simulink model "ASM_Traffic_new"  (R2024a)
settings: Solver=ode1  StartTime=SIM.tstart.v  StopTime=SIM.tend.v  FixedStep=SIM.StepSize.v  RelTol=1e-3
PostLoadFcn:
  | if any(exist('dsrtsu_mdlpostloadfcn', 'file') ~= 0), dsrtsu_mdlpostloadfcn('Execute', bdroot); end
  | try, asm_mdl_postloadfcn(bdroot, 'UpdateModel', 3600); catch, disp(lasterr); end,
InitFcn:
  | , if any(exist('rtifpga_mdlclblib', 'file') ~= 0), rtifpga_mdlclblib('Init', bdroot); end,
  | , if any(exist('dsmpb_private', 'file') ~= 0), dsmpb_private('dsmpb_mdlclblib', 'Init', bdroot); end,
undefined symbols (not defined in the file): _to_, a0b2, ASM_BrakeHydraulics_DemoSystems, ASM_VehicleDynamics_DemoSystems, b98103fe8ad365046cd0, BrakeCircuit, CPT, Crankshaft, DiscIntNeverNeededParam, dsmsi, FinalDriveAssembly, MDL, ModeSignals, Pos_BrakePedal_Maneuver, rad, RefSignals, s_to_rpm, SIM, SoftECU, Suspension, Tire, Transmission
libraries: ASM_Traffic_lib x135, simulink x100, ASM_Utils_lib x77, ASM_VehicleDynamics_lib x70, ASM_Environment_lib x22, dsmpblib x20, dsmsilib x15, MDLD_Utils_lib x10, ASM_BrakeHydraulics_lib x3
(part 54 of 63)

== system ASM_Traffic_new/VehicleDynamics/Plant/VehicleDynamics/VehicleMovement/ASMSignalCollector/Vehicle_Movement_Info_Car ==
  Reset[] : Inport
  CoGAndWheelVelocities : Inport  Port=2
  ASMBUS_VehicleDynamics_CoordinateTransformation : Inport  Port=3
  ASMBUS_VehicleDynamics_VehicleMotion : Inport  Port=4
  ASMBUS_VehicleDynamics_MassForcesAndTorques : Inport  Port=5
  ASMBUS_VehicleDynamics_VehicleMass : Inport  Port=6
  ASMBUS_VehicleDynamics_SensorMotion : Inport  Port=7
  ASMBUS_VehicleDynamics_Suspension : Inport  Port=8
  ASMBUS_VehicleDynamics_Steering : Inport  Port=9
  Accelerations : Subsystem
  Bus Selector : BusSelector  OutputSignals=GeneralizedVelocitiesDerivative.v_Vehicle_dt[x;y;z][m|s2],GeneralizedVelocitiesDerivative.w_Vehicle_dt[x;y;z][rad|s2],GeneralizedVelocitiesDerivative.q_Wheel_dt2[q1_Front;q2_Front;q1_Rear;q2_Rear][],GeneralizedVelocities.v_Vehicle[x;y;z][m|s],GeneralizedVelocities.w_Vehicle[x;y;z][rad|s],GeneralizedVelocities.q_Wheel_dt[q1_Front;q2_Front;q1_Rear;q2_Rear][],GeneralizedForcesAndTorques,GeneralizedVelocitiesDerivative
  Bus Selector1 : BusSelector  OutputSignals=VehiclePositionCoorSysE.Pos_Vehicle_CoorSys_E[x;y;z][m],VehiclePositionCoorSysE.Angle_V[Alpha;Beta;Gamma][deg],WheelPositionCoorSysE.Pos_FL_Wheels_CoorSys_E[x;y;z][m],WheelPositionCoorSysE.Pos_FR_Wheels_CoorSys_E[x;y;z][m],WheelPositionCoorSysE.Pos_RL_Wheels_CoorSys_E[x;y;z][m],WheelPositionCoorSysE.Pos_RR_Wheels_CoorSys_E[x;y;z][m],RotationMatrix_V_to_E[3x3],RotationMatrix_V_to_E_T[3x3],a_Gravity_CoorSys_V[x;y;z][m|s2]
  BusCreator2 : BusCreator  Inputs=8
  CoordinateTransformation : Subsystem
  Positions : Subsystem
  VehicleEquationOfMotion : Subsystem
  Velocities : Subsystem
  ASMSignalBus : Outport  VectorParamsAs1DForOutWhenUnconnected=off
  wires:
  Bus Selector1/1 -> Positions/3(Pos_Vehicle_CoorSys_E[x;y;z][m])  "<Pos_Vehicle_CoorSys_E[x;y;z][m]>"
  ASMBUS_VehicleDynamics_MassForcesAndTorques/1 -> BusCreator2/8, Accelerations/1(ASMBUS_VehicleDynamics_MassForcesAndTorques)
  Velocities/1(Velocities) -> Positions/1(Velocities), BusCreator2/2
  Bus Selector/3 -> Accelerations/8(q_Wheel_dt2[q1_Front;q2_Front;q1_Rear;q2_Rear][])  "<q_Wheel_dt2[q1_Front;q2_Front;q1_Rear;q2_Rear][]>"
  Bus Selector1/7 -> Positions/9(RotationMatrix_V_to_E[3x3])  "<RotationMatrix_V_to_E[3x3]>"
  Bus Selector1/9 -> Accelerations/5(a_Gravity_CoorSys_V[x;y;z][m|s2]), CoordinateTransformation/1(a_Gravity_CoorSys_V[x;y;z][m|s2])  "<a_Gravity_CoorSys_V[x;y;z][m|s2]>"
  Bus Selector1/2 -> Positions/4(Angle_V[Alpha;Beta;Gamma][deg])  "<Angle_V[Alpha;Beta;Gamma][deg]>"
  Bus Selector/2 -> Accelerations/7(w_Vehicle_dt[x;y;z][rad|s2])  "<w_Vehicle_dt[x;y;z][rad|s2]>"
  ASMBUS_VehicleDynamics_CoordinateTransformation/1 -> Bus Selector1/1
  Bus Selector/6 -> Velocities/4(q_Wheel_dt[q1_Front;q2_Front;q1_Rear;q2_Rear][])  "<q_Wheel_dt[q1_Front;q2_Front;q1_Rear;q2_Rear][]>"
  Bus Selector/7 -> VehicleEquationOfMotion/1(GeneralizedForcesAndTorques)  "<GeneralizedForcesAndTorques>"
  ASMBUS_VehicleDynamics_SensorMotion/1 -> BusCreator2/6
  Bus Selector1/5 -> Positions/7(Pos_RL_Wheels_CoorSys_E[x;y;z][m])  "<Pos_RL_Wheels_CoorSys_E[x;y;z][m]>"
  Positions/1(Positions) -> BusCreator2/3
  VehicleEquationOfMotion/1(VehicleEquationOfMotion) -> BusCreator2/4
  Accelerations/1(Accelerations) -> BusCreator2/1
  ASMBUS_VehicleDynamics_VehicleMass/1 -> BusCreator2/7, Accelerations/2(ASMBUS_VehicleDynamics_VehicleMass)
  ASMBUS_VehicleDynamics_VehicleMotion/1 -> Bus Selector/1
  Bus Selector1/4 -> Positions/6(Pos_FR_Wheels_CoorSys_E[x;y;z][m])  "<Pos_FR_Wheels_CoorSys_E[x;y;z][m]>"
  ASMBUS_VehicleDynamics_Steering/1 -> Accelerations/4(ASMBUS_VehicleDynamics_Steering)
  Bus Selector/5 -> Velocities/3(w_Vehicle[x;y;z][rad|s])  "<w_Vehicle[x;y;z][rad|s]>"
  Bus Selector/8 -> VehicleEquationOfMotion/2(GeneralizedVelocitiesDerivative)  "<GeneralizedVelocitiesDerivative>"
  CoordinateTransformation/1(CoordinateTransformation) -> BusCreator2/5
  Bus Selector/1 -> Accelerations/6(v_Vehicle_dt[x;y;z][m|s2])  "<v_Vehicle_dt[x;y;z][m|s2]>"
  BusCreator2/1 -> ASMSignalBus/1  "VehicleMovement"
  Bus Selector1/6 -> Positions/8(Pos_RR_Wheels_CoorSys_E[x;y;z][m])  "<Pos_RR_Wheels_CoorSys_E[x;y;z][m]>"
  Bus Selector1/3 -> Positions/5(Pos_FL_Wheels_CoorSys_E[x;y;z][m])  "<Pos_FL_Wheels_CoorSys_E[x;y;z][m]>"
  ASMBUS_VehicleDynamics_Suspension/1 -> Accelerations/3(ASMBUS_VehicleDynamics_Suspension)
  Reset[]/1 -> Positions/2(Reset[])
  CoGAndWheelVelocities/1 -> Velocities/1(CoGAndWheelVelocities)
  Bus Selector1/8 -> Positions/10(RotationMatrix_V_to_E_T[3x3])  "<RotationMatrix_V_to_E_T[3x3]>"
  Bus Selector/4 -> Velocities/2(v_Vehicle[x;y;z][m|s])  "<v_Vehicle[x;y;z][m|s]>"

== system ASM_Traffic_new/AnimationInterface/ANIMATION_INTERFACE/Sensors/Object_Sensor_2D_Points/Calc_Object_Sensor_2D_Points/Sensor_Points/ForIterator_Current ==
  dim_animation_point[] : Inport
  init_animation_point[] : Inport  Port=2
  num_sensor_rays[] : Inport  Port=3
  distance_sensor_out : Inport  Port=4
  angle_sensor_out : Inport  Port=5
  Add1 : Sum  Inputs=+-
  AnimationPoint_Idx : MultiPortSwitch  DataPortOrder=Zero-based contiguous  Inputs=2  zeroidx=on  SaturateOnIntegerOverflow=off  InputSameDT=off
  Assignment_Angle : Assignment  IndexOptions=Index vector (port)  Indices=1  OutputSizes=1
  Assignment_Distance : Assignment  IndexOptions=Index vector (port)  Indices=1  OutputSizes=1
  Calc_Output_Idx[] : Sum
  Calc_Saturated_Iteration_Idx : simulink/Discontinuities/Saturation Dynamic  OutMin=[]  OutMax=[]  OutDataTypeStr=Inherit: Same as second input  OutDataType=fixdt(1, 16)  OutScaling=2^-10  DoSatur=off
  Calc_Scaling_Step : Rounding  Operator=ceil
  Constant1 : Constant
  Constant2 : Constant
  Default_Idx : Constant
  Default_Value : Constant  Value=0
  Divide : Product  Inputs=*/
  For Iterator : ForIterator  ResetStates=reset  IterationSource=external  IterationLimit=36
  Iteration_Idx_LowBound : Constant
  Iteration_Idx_UpBound : MultiPortSwitch  DataPortOrder=Zero-based contiguous  Inputs=2  zeroidx=on  SaturateOnIntegerOverflow=off  InputSameDT=off
  Multiport Switch : MultiPortSwitch  DataPortOrder=Zero-based contiguous  Inputs=2  zeroidx=on  SaturateOnIntegerOverflow=off  InputSameDT=off
  Output_Idx : MultiPortSwitch  DataPortOrder=Zero-based contiguous  Inputs=2  zeroidx=on  SaturateOnIntegerOverflow=off  InputSameDT=off
  Point_Is_Unused : Constant  Value=0
  Product : Product
  Relational Operator : RelationalOperator  Operator=<=  OutDataTypeStr=boolean  InputSameDT=off
  Relational Operator1 : RelationalOperator  Operator=<  OutDataTypeStr=boolean  InputSameDT=off
  Relational Operator2 : RelationalOperator  Operator=<  OutDataTypeStr=boolean  InputSameDT=off
  Relational Operator3 : RelationalOperator  Operator=>  OutDataTypeStr=boolean  InputSameDT=off
  Saturate_to_sensor_output_dim : Saturate  UpperLimit=MDL.Traffic.Sensors.ObjectSensor2D_Calculation.Const_Sensor_Output_Dimension.v  LowerLimit=1
  Select_Angle : Selector  InputPortWidth=MDL.Traffic.Sensors.ObjectSensor2D_Calculation.Const_Sensor_Output_Dimension.v  IndexOptions=Starting index (port)  Indices=[1 3]  OutputSizes=1
  Select_Default_Angle : MultiPortSwitch  DataPortOrder=Zero-based contiguous  Inputs=2  zeroidx=on  SaturateOnIntegerOverflow=off  InputSameDT=off
  Select_Default_Distance : MultiPortSwitch  DataPortOrder=Zero-based contiguous  Inputs=2  zeroidx=on  SaturateOnIntegerOverflow=off  InputSameDT=off
  Select_Distance : Selector  InputPortWidth=MDL.Traffic.Sensors.ObjectSensor2D_Calculation.Const_Sensor_Output_Dimension.v  IndexOptions=Starting index (port)  Indices=[1 3]  OutputSizes=1
  distance_animation_point[m] : Outport  InitialOutput=0  VectorParamsAs1DForOutWhenUnconnected=off
  angle_animation_point[deg] : Outport  Port=2  InitialOutput=0  VectorParamsAs1DForOutWhenUnconnected=off
  flag_point_used[0|1] : Outport  Port=3  InitialOutput=0  VectorParamsAs1DForOutWhenUnconnected=off
  wires:
  Point_Is_Unused/1 -> Relational Operator3/2
  Saturate_to_sensor_output_dim/1 -> Relational Operator/1, Iteration_Idx_UpBound/3, Relational Operator1/1, Divide/1, Relational Operator2/1
  init_animation_point[]/1 -> Assignment_Distance/1, Assignment_Angle/1
  Assignment_Distance/1 -> distance_animation_point[m]/1, Relational Operator3/1
  Assignment_Angle/1 -> angle_animation_point[deg]/1
  angle_sensor_out/1 -> Select_Angle/1
  distance_sensor_out/1 -> Select_Distance/1
  Select_Distance/1 -> Select_Default_Distance/2
  Select_Angle/1 -> Select_Default_Angle/2
  Relational Operator/1 -> Multiport Switch/1
  Output_Idx/1 -> Multiport Switch/2
  Multiport Switch/1 -> Select_Angle/2, Select_Distance/2
  AnimationPoint_Idx/1 -> Multiport Switch/3, Assignment_Angle/3, Assignment_Distance/3
  For Iterator/1 -> Calc_Saturated_Iteration_Idx/2
  Iteration_Idx_LowBound/1 -> Calc_Saturated_Iteration_Idx/3
  Iteration_Idx_UpBound/1 -> Calc_Saturated_Iteration_Idx/1
  Relational Operator1/1 -> Iteration_Idx_UpBound/1
  Relational Operator2/1 -> AnimationPoint_Idx/1, Output_Idx/1, Select_Default_Distance/1, Select_Default_Angle/1
  Default_Idx/1 -> AnimationPoint_Idx/3, Output_Idx/3
  Calc_Output_Idx[]/1 -> Output_Idx/2, Relational Operator2/2
  Add1/1 -> Product/2
  Constant2/1 -> Calc_Output_Idx[]/2
  Product/1 -> Calc_Output_Idx[]/1
  Constant1/1 -> Add1/2
  Calc_Scaling_Step/1 -> Product/1
  Calc_Saturated_Iteration_Idx/1 -> Add1/1, AnimationPoint_Idx/2
  Divide/1 -> Calc_Scaling_Step/1
  dim_animation_point[]/1 -> For Iterator/1, Iteration_Idx_UpBound/2, Relational Operator1/2, Divide/2, Relational Operator/2
  num_sensor_rays[]/1 -> Saturate_to_sensor_output_dim/1
  Select_Default_Distance/1 -> Assignment_Distance/2
  Default_Value/1 -> Select_Default_Distance/3, Select_Default_Angle/3
  Select_Default_Angle/1 -> Assignment_Angle/2
  Relational Operator3/1 -> flag_point_used[0|1]/1

== system ASM_Traffic_new/DomainControl/DriverAssistance/Control/SoftECU_ACC/Soft_ECU_ACC/Map_Inputs/Maneuver ==
  note: Initial value is set
      | to AEBOff (3)
  ECU_Commands[] : Inport
  Reset[0|1] : Inport  Port=2
  ACC_BrakeMode_Default : Constant  Value=3
  Add : Sum  Inputs=+++
  Fcn1 : Fcn  Expr=u(1)==1020
  Fcn10 : Fcn  Expr=u(1)==1031
  Fcn2 : Fcn  Expr=u(1)==1030
  Fcn3 : Fcn  Expr=u(1)==1022
  Fcn4 : Fcn  Expr=u(1)==1021
  Fcn5 : Fcn  Expr=u(1)==1013
  Fcn6 : Fcn  Expr=u(1)==1011
  Fcn7 : Fcn  Expr=u(1)==1010
  Fcn8 : Fcn  Expr=u(1)==1012
  Fcn9 : Fcn  Expr=u(1)==1032
  Gain : Gain
  Gain1 : Gain  Gain=2
  Gain2 : Gain  Gain=3
  Logical Operator : Logic  Operator=OR  Inputs=4  AllPortsSameDT=off  OutDataTypeStr=boolean
  Memory : Memory  InitialCondition=3
  Switch : Switch  Threshold=0.5  SaturateOnIntegerOverflow=off  InputSameDT=off
  Switch1 : Switch  Threshold=0.5  SaturateOnIntegerOverflow=off  InputSameDT=off
  pos_edge_detection : Subsystem
  pos_edge_detection1 : Subsystem
  pos_edge_detection2 : Subsystem
  pos_edge_detection3 : Subsystem
  Sw_ACC_On[0Off|1On] : Outport  VectorParamsAs1DForOutWhenUnconnected=off
  Sw_ACC_Off[0Off|1On] : Outport  Port=2  VectorParamsAs1DForOutWhenUnconnected=off
  Sw_ACC_Cancel[0Off|1On] : Outport  Port=3  VectorParamsAs1DForOutWhenUnconnected=off
  Sw_ACC_Resume[0Off|1On] : Outport  Port=4  VectorParamsAs1DForOutWhenUnconnected=off
  Sw_ACC_Speed_Set[0Off|1On] : Outport  Port=5  VectorParamsAs1DForOutWhenUnconnected=off
  Sw_ACC_Speed_Increase[0Off|1On] : Outport  Port=6  VectorParamsAs1DForOutWhenUnconnected=off
  Sw_ACC_Speed_Decrease[0Off|1On] : Outport  Port=7  VectorParamsAs1DForOutWhenUnconnected=off
  Sw_ACC_BrakeMode[1Comfort|2AEBOnly|3AEBOff] : Outport  Port=8  VectorParamsAs1DForOutWhenUnconnected=off
  wires:
  ACC_BrakeMode_Default/1 -> Switch1/1
  Switch1/1 -> Switch/1
  Reset[0|1]/1 -> pos_edge_detection3/1(In1)
  Add/1 -> Switch1/3
  pos_edge_detection3/1(Out1) -> Logical Operator/4, Switch1/2
  Memory/1 -> Switch/3
  Switch/1 -> Memory/1, Sw_ACC_BrakeMode[1Comfort|2AEBOnly|3AEBOff]/1
  Logical Operator/1 -> Switch/2
  Gain/1 -> Add/1
  Gain1/1 -> Add/2
  Gain2/1 -> Add/3
  pos_edge_detection2/1(Out1) -> Logical Operator/3
  pos_edge_detection1/1(Out1) -> Logical Operator/2
  pos_edge_detection/1(Out1) -> Logical Operator/1
  Fcn2/1 -> Gain/1, pos_edge_detection2/1(In1)
  Fcn10/1 -> Gain1/1, pos_edge_detection1/1(In1)
  Fcn9/1 -> Gain2/1, pos_edge_detection/1(In1)
  ECU_Commands[]/1 -> Fcn3/1, Fcn2/1, Fcn10/1, Fcn9/1, Fcn4/1, Fcn1/1, Fcn5/1, Fcn8/1, Fcn6/1, Fcn7/1
  Fcn1/1 -> Sw_ACC_Speed_Set[0Off|1On]/1
  Fcn8/1 -> Sw_ACC_Cancel[0Off|1On]/1
  Fcn5/1 -> Sw_ACC_Resume[0Off|1On]/1
  Fcn4/1 -> Sw_ACC_Speed_Increase[0Off|1On]/1
  Fcn3/1 -> Sw_ACC_Speed_Decrease[0Off|1On]/1
  Fcn7/1 -> Sw_ACC_On[0Off|1On]/1
  Fcn6/1 -> Sw_ACC_Off[0Off|1On]/1

== system ASM_Traffic_new/Drivetrain/Plant/Drivetrain/Final_Drive_Assembly/ASMSignalCollector/Clutch_4WD/Clutch_4WD ==
  Bus Selector1 : BusSelector  OutputSignals=omega_Clutch_4WD_In[rad|s],Trq_Lock_Clutch_4WD[Nm],omega_Clutch_4WD_Out[rad|s]
  BusCreator1 : BusCreator  Inputs=3
  Out : Outport  VectorParamsAs1DForOutWhenUnconnected=off
  wires:
  Bus Selector1/2 -> BusCreator1/2  "<Trq_Lock_Clutch_4WD[Nm]>"
  [ASMBUS_Drivetrain_Clutch_4WD] -> Bus Selector1/1
  Bus Selector1/1 -> BusCreator1/1  "<omega_Clutch_4WD_In[rad|s]>"
  BusCreator1/1 -> Out/1  "Clutch_4WD"
  Bus Selector1/3 -> BusCreator1/3  "<omega_Clutch_4WD_Out[rad|s]>"

== system ASM_Traffic_new/Drivetrain/Plant/Drivetrain/Final_Drive_Assembly/ASMSignalCollector/Clutch_4WD/Dummy_Clutch_4WD ==
  BusCreator : BusCreator  Inputs=3
  Dummy_Trq_Lock_Clutch_4WD : Constant  Value=0
  Dummy_omega_Clutch_4WD_In : Constant  Value=0
  Dummy_omega_Clutch_4WD_Out : Constant  Value=0
  Out : Outport  VectorParamsAs1DForOutWhenUnconnected=off
  wires:
  Dummy_Trq_Lock_Clutch_4WD/1 -> BusCreator/2  "Trq_Lock_Clutch_4WD[Nm]"
  BusCreator/1 -> Out/1  "Clutch_4WD"
  Dummy_omega_Clutch_4WD_Out/1 -> BusCreator/3  "omega_Clutch_4WD_Out[rad|s]"
  Dummy_omega_Clutch_4WD_In/1 -> BusCreator/1  "omega_Clutch_4WD_In[rad|s]"

== system ASM_Traffic_new/Drivetrain/Plant/Drivetrain/Final_Drive_Assembly/ASMSignalCollector/Shaft_CF/Dummy_CF_Shaft ==
  BusCreator1 : BusCreator  Inputs=1
  Dummy_Trq_CF_Shaft[Nm] : Constant  Value=0
  Out : Outport  VectorParamsAs1DForOutWhenUnconnected=off
  wires:
  Dummy_Trq_CF_Shaft[Nm]/1 -> BusCreator1/1  "Trq_CF_Shaft[Nm]"
  BusCreator1/1 -> Out/1  "Shaft_CF"

== system ASM_Traffic_new/Drivetrain/Plant/Drivetrain/Final_Drive_Assembly/ASMSignalCollector/Shaft_CR/Dummy_CR_Shaft ==
  BusCreator1 : BusCreator  Inputs=1
  Dummy_Trq_CR_Shaft : Constant  Value=0
  Out : Outport  VectorParamsAs1DForOutWhenUnconnected=off
  wires:
  BusCreator1/1 -> Out/1  "Shaft_CR"
  Dummy_Trq_CR_Shaft/1 -> BusCreator1/1  "Trq_CR_Shaft[Nm]"

== system ASM_Traffic_new/Drivetrain/Plant/Drivetrain/Final_Drive_Assembly/ASMSignalCollector/Transfer_Gearbox/Dummy_Transfer_Gearbox ==
  BusCreator : BusCreator  Inputs=2
  Dummy_Trq_Cage : Constant  Value=0
  Dummy_omega_Shaft : Constant  Value=0
  Out : Outport  VectorParamsAs1DForOutWhenUnconnected=off
  wires:
  Dummy_omega_Shaft/1 -> BusCreator/2  "omega_Shaft[rad|s]"
  BusCreator/1 -> Out/1  "TransferGearbox"
  Dummy_Trq_Cage/1 -> BusCreator/1  "Trq_Cage[Nm]"

== system ASM_Traffic_new/Drivetrain/Plant/Drivetrain/Final_Drive_Assembly/ASMSignalCollector/Transfer_Gearbox/Transfer_Gearbox ==
  Bus Selector1 : BusSelector  OutputSignals=Trq_Cage[Nm],omega_Shaft[rad|s]
  BusCreator : BusCreator  Inputs=2
  Out : Outport  VectorParamsAs1DForOutWhenUnconnected=off
  wires:
  Bus Selector1/2 -> BusCreator/2  "<omega_Shaft[rad|s]>"
  Bus Selector1/1 -> BusCreator/1  "<Trq_Cage[Nm]>"
  BusCreator/1 -> Out/1  "TransferGearbox"
  [ASMBUS_Drivetrain_Transfer_Gearbox] -> Bus Selector1/1

== system ASM_Traffic_new/Environment/GroundTruth/UserInterface/PAR_Plant/Ego_Vehicle/Indicator_State[]/ASM_OSI_Mapping ==
  ASM_Vehicle_TurnLights[] : Inport
  Table_ASM_To_OSI : Lookup_n-D  NumberOfTableDimensions=1  BreakpointsForDimension1=[0,1,2,3]  Table=[2,3,4,5]  InterpMethod=Nearest  InternalRulePriority=Speed  RndMeth=Simplest
  Indicator_State[] : Outport  VectorParamsAs1DForOutWhenUnconnected=off
  wires:
  Table_ASM_To_OSI/1 -> Indicator_State[]/1
  ASM_Vehicle_TurnLights[]/1 -> Table_ASM_To_OSI/1

== system ASM_Traffic_new/Environment/GroundTruth/UserInterface/PAR_Plant/Fellow_Vehicles/Lightstates_Fellow1/Indicator_State[] ==
  Fellow_TurnLights[] : Inport
  ASM_OSI_Mapping : Subsystem
  Ext_Indicator_State[] : Constant  Value=0
  Multiport Switch : MultiPortSwitch  DataPortOrder=Zero-based contiguous  zeroidx=on  SaturateOnIntegerOverflow=off  InputSameDT=off
  Rounding Function : Rounding  Operator=round
  Saturation : Saturate  UpperLimit=2  LowerLimit=0
  Stim_Indicator_State[] : Constant  Value=0
  Sw_Indicator[0Stim|1Ext|2Mnv] : Constant  Value=2
  Indicator_State[] : Outport  VectorParamsAs1DForOutWhenUnconnected=off
  wires:
  ASM_OSI_Mapping/1(Indicator_State[]) -> Multiport Switch/4  "Mnv_Indicator_State[]"
  Stim_Indicator_State[]/1 -> Multiport Switch/2  "Stim_Indicator_State[]"
  Multiport Switch/1 -> Indicator_State[]/1  "Indicator_State[]"
  Saturation/1 -> Multiport Switch/1
  Rounding Function/1 -> Saturation/1
  Ext_Indicator_State[]/1 -> Multiport Switch/3  "Ext_Indicator_State[]"
  Fellow_TurnLights[]/1 -> ASM_OSI_Mapping/1(Fellow_TurnLights[])
  Sw_Indicator[0Stim|1Ext|2Mnv]/1 -> Rounding Function/1  "Sw_Indicator[0Stim|1Ext|2Mnv]"

== system ASM_Traffic_new/Environment/GroundTruth/UserInterface/PAR_Plant/Fellow_Vehicles/Lightstates_Fellow10/Indicator_State[] ==
  Fellow_TurnLights[] : Inport
  ASM_OSI_Mapping : Subsystem
  Ext_Indicator_State[] : Constant  Value=0
  Multiport Switch : MultiPortSwitch  DataPortOrder=Zero-based contiguous  zeroidx=on  SaturateOnIntegerOverflow=off  InputSameDT=off
  Rounding Function : Rounding  Operator=round
  Saturation : Saturate  UpperLimit=2  LowerLimit=0
  Stim_Indicator_State[] : Constant  Value=0
  Sw_Indicator[0Stim|1Ext|2Mnv] : Constant  Value=2
  Indicator_State[] : Outport  VectorParamsAs1DForOutWhenUnconnected=off
  wires:
  Sw_Indicator[0Stim|1Ext|2Mnv]/1 -> Rounding Function/1  "Sw_Indicator[0Stim|1Ext|2Mnv]"
  Fellow_TurnLights[]/1 -> ASM_OSI_Mapping/1(Fellow_TurnLights[])
  Ext_Indicator_State[]/1 -> Multiport Switch/3  "Ext_Indicator_State[]"
  Rounding Function/1 -> Saturation/1
  Saturation/1 -> Multiport Switch/1
  Multiport Switch/1 -> Indicator_State[]/1  "Indicator_State[]"
  Stim_Indicator_State[]/1 -> Multiport Switch/2  "Stim_Indicator_State[]"
  ASM_OSI_Mapping/1(Indicator_State[]) -> Multiport Switch/4  "Mnv_Indicator_State[]"

== system ASM_Traffic_new/Environment/GroundTruth/UserInterface/PAR_Plant/Fellow_Vehicles/Lightstates_Fellow11/Indicator_State[] ==
  Fellow_TurnLights[] : Inport
  ASM_OSI_Mapping : Subsystem
  Ext_Indicator_State[] : Constant  Value=0
  Multiport Switch : MultiPortSwitch  DataPortOrder=Zero-based contiguous  zeroidx=on  SaturateOnIntegerOverflow=off  InputSameDT=off
  Rounding Function : Rounding  Operator=round
  Saturation : Saturate  UpperLimit=2  LowerLimit=0
  Stim_Indicator_State[] : Constant  Value=0
  Sw_Indicator[0Stim|1Ext|2Mnv] : Constant  Value=2
  Indicator_State[] : Outport  VectorParamsAs1DForOutWhenUnconnected=off
  wires:
  ASM_OSI_Mapping/1(Indicator_State[]) -> Multiport Switch/4  "Mnv_Indicator_State[]"
  Stim_Indicator_State[]/1 -> Multiport Switch/2  "Stim_Indicator_State[]"
  Multiport Switch/1 -> Indicator_State[]/1  "Indicator_State[]"
  Saturation/1 -> Multiport Switch/1
  Rounding Function/1 -> Saturation/1
  Ext_Indicator_State[]/1 -> Multiport Switch/3  "Ext_Indicator_State[]"
  Fellow_TurnLights[]/1 -> ASM_OSI_Mapping/1(Fellow_TurnLights[])
  Sw_Indicator[0Stim|1Ext|2Mnv]/1 -> Rounding Function/1  "Sw_Indicator[0Stim|1Ext|2Mnv]"

== system ASM_Traffic_new/Environment/GroundTruth/UserInterface/PAR_Plant/Fellow_Vehicles/Lightstates_Fellow12/Indicator_State[] ==
  Fellow_TurnLights[] : Inport
  ASM_OSI_Mapping : Subsystem
  Ext_Indicator_State[] : Constant  Value=0
  Multiport Switch : MultiPortSwitch  DataPortOrder=Zero-based contiguous  zeroidx=on  SaturateOnIntegerOverflow=off  InputSameDT=off
  Rounding Function : Rounding  Operator=round
  Saturation : Saturate  UpperLimit=2  LowerLimit=0
  Stim_Indicator_State[] : Constant  Value=0
  Sw_Indicator[0Stim|1Ext|2Mnv] : Constant  Value=2
  Indicator_State[] : Outport  VectorParamsAs1DForOutWhenUnconnected=off
  wires:
  Sw_Indicator[0Stim|1Ext|2Mnv]/1 -> Rounding Function/1  "Sw_Indicator[0Stim|1Ext|2Mnv]"
  Fellow_TurnLights[]/1 -> ASM_OSI_Mapping/1(Fellow_TurnLights[])
  Ext_Indicator_State[]/1 -> Multiport Switch/3  "Ext_Indicator_State[]"
  Rounding Function/1 -> Saturation/1
  Saturation/1 -> Multiport Switch/1
  Multiport Switch/1 -> Indicator_State[]/1  "Indicator_State[]"
  Stim_Indicator_State[]/1 -> Multiport Switch/2  "Stim_Indicator_State[]"
  ASM_OSI_Mapping/1(Indicator_State[]) -> Multiport Switch/4  "Mnv_Indicator_State[]"

== system ASM_Traffic_new/Environment/GroundTruth/UserInterface/PAR_Plant/Fellow_Vehicles/Lightstates_Fellow13/Indicator_State[] ==
  Fellow_TurnLights[] : Inport
  ASM_OSI_Mapping : Subsystem
  Ext_Indicator_State[] : Constant  Value=0
  Multiport Switch : MultiPortSwitch  DataPortOrder=Zero-based contiguous  zeroidx=on  SaturateOnIntegerOverflow=off  InputSameDT=off
  Rounding Function : Rounding  Operator=round
  Saturation : Saturate  UpperLimit=2  LowerLimit=0
  Stim_Indicator_State[] : Constant  Value=0
  Sw_Indicator[0Stim|1Ext|2Mnv] : Constant  Value=2
  Indicator_State[] : Outport  VectorParamsAs1DForOutWhenUnconnected=off
  wires:
  ASM_OSI_Mapping/1(Indicator_State[]) -> Multiport Switch/4  "Mnv_Indicator_State[]"
  Stim_Indicator_State[]/1 -> Multiport Switch/2  "Stim_Indicator_State[]"
  Multiport Switch/1 -> Indicator_State[]/1  "Indicator_State[]"
  Saturation/1 -> Multiport Switch/1
  Rounding Function/1 -> Saturation/1
  Ext_Indicator_State[]/1 -> Multiport Switch/3  "Ext_Indicator_State[]"
  Fellow_TurnLights[]/1 -> ASM_OSI_Mapping/1(Fellow_TurnLights[])
  Sw_Indicator[0Stim|1Ext|2Mnv]/1 -> Rounding Function/1  "Sw_Indicator[0Stim|1Ext|2Mnv]"

== system ASM_Traffic_new/Environment/GroundTruth/UserInterface/PAR_Plant/Fellow_Vehicles/Lightstates_Fellow14/Indicator_State[] ==
  Fellow_TurnLights[] : Inport
  ASM_OSI_Mapping : Subsystem
  Ext_Indicator_State[] : Constant  Value=0
  Multiport Switch : MultiPortSwitch  DataPortOrder=Zero-based contiguous  zeroidx=on  SaturateOnIntegerOverflow=off  InputSameDT=off
  Rounding Function : Rounding  Operator=round
  Saturation : Saturate  UpperLimit=2  LowerLimit=0
  Stim_Indicator_State[] : Constant  Value=0
  Sw_Indicator[0Stim|1Ext|2Mnv] : Constant  Value=2
  Indicator_State[] : Outport  VectorParamsAs1DForOutWhenUnconnected=off
  wires:
  Sw_Indicator[0Stim|1Ext|2Mnv]/1 -> Rounding Function/1  "Sw_Indicator[0Stim|1Ext|2Mnv]"
  Fellow_TurnLights[]/1 -> ASM_OSI_Mapping/1(Fellow_TurnLights[])
  Ext_Indicator_State[]/1 -> Multiport Switch/3  "Ext_Indicator_State[]"
  Rounding Function/1 -> Saturation/1
  Saturation/1 -> Multiport Switch/1
  Multiport Switch/1 -> Indicator_State[]/1  "Indicator_State[]"
  Stim_Indicator_State[]/1 -> Multiport Switch/2  "Stim_Indicator_State[]"
  ASM_OSI_Mapping/1(Indicator_State[]) -> Multiport Switch/4  "Mnv_Indicator_State[]"

== system ASM_Traffic_new/Environment/GroundTruth/UserInterface/PAR_Plant/Fellow_Vehicles/Lightstates_Fellow15/Indicator_State[] ==
  Fellow_TurnLights[] : Inport
  ASM_OSI_Mapping : Subsystem
  Ext_Indicator_State[] : Constant  Value=0
  Multiport Switch : MultiPortSwitch  DataPortOrder=Zero-based contiguous  zeroidx=on  SaturateOnIntegerOverflow=off  InputSameDT=off
  Rounding Function : Rounding  Operator=round
  Saturation : Saturate  UpperLimit=2  LowerLimit=0
  Stim_Indicator_State[] : Constant  Value=0
  Sw_Indicator[0Stim|1Ext|2Mnv] : Constant  Value=2
  Indicator_State[] : Outport  VectorParamsAs1DForOutWhenUnconnected=off
  wires:
  ASM_OSI_Mapping/1(Indicator_State[]) -> Multiport Switch/4  "Mnv_Indicator_State[]"
  Stim_Indicator_State[]/1 -> Multiport Switch/2  "Stim_Indicator_State[]"
  Multiport Switch/1 -> Indicator_State[]/1  "Indicator_State[]"
  Saturation/1 -> Multiport Switch/1
  Rounding Function/1 -> Saturation/1
  Ext_Indicator_State[]/1 -> Multiport Switch/3  "Ext_Indicator_State[]"
  Fellow_TurnLights[]/1 -> ASM_OSI_Mapping/1(Fellow_TurnLights[])
  Sw_Indicator[0Stim|1Ext|2Mnv]/1 -> Rounding Function/1  "Sw_Indicator[0Stim|1Ext|2Mnv]"

== system ASM_Traffic_new/Environment/GroundTruth/UserInterface/PAR_Plant/Fellow_Vehicles/Lightstates_Fellow16/Indicator_State[] ==
  Fellow_TurnLights[] : Inport
  ASM_OSI_Mapping : Subsystem
  Ext_Indicator_State[] : Constant  Value=0
  Multiport Switch : MultiPortSwitch  DataPortOrder=Zero-based contiguous  zeroidx=on  SaturateOnIntegerOverflow=off  InputSameDT=off
  Rounding Function : Rounding  Operator=round
  Saturation : Saturate  UpperLimit=2  LowerLimit=0
  Stim_Indicator_State[] : Constant  Value=0
  Sw_Indicator[0Stim|1Ext|2Mnv] : Constant  Value=2
  Indicator_State[] : Outport  VectorParamsAs1DForOutWhenUnconnected=off
  wires:
  Sw_Indicator[0Stim|1Ext|2Mnv]/1 -> Rounding Function/1  "Sw_Indicator[0Stim|1Ext|2Mnv]"
  Fellow_TurnLights[]/1 -> ASM_OSI_Mapping/1(Fellow_TurnLights[])
  Ext_Indicator_State[]/1 -> Multiport Switch/3  "Ext_Indicator_State[]"
  Rounding Function/1 -> Saturation/1
  Saturation/1 -> Multiport Switch/1
  Multiport Switch/1 -> Indicator_State[]/1  "Indicator_State[]"
  Stim_Indicator_State[]/1 -> Multiport Switch/2  "Stim_Indicator_State[]"
  ASM_OSI_Mapping/1(Indicator_State[]) -> Multiport Switch/4  "Mnv_Indicator_State[]"

== system ASM_Traffic_new/Environment/GroundTruth/UserInterface/PAR_Plant/Fellow_Vehicles/Lightstates_Fellow17/Indicator_State[] ==
  Fellow_TurnLights[] : Inport
  ASM_OSI_Mapping : Subsystem
  Ext_Indicator_State[] : Constant  Value=0
  Multiport Switch : MultiPortSwitch  DataPortOrder=Zero-based contiguous  zeroidx=on  SaturateOnIntegerOverflow=off  InputSameDT=off
  Rounding Function : Rounding  Operator=round
  Saturation : Saturate  UpperLimit=2  LowerLimit=0
  Stim_Indicator_State[] : Constant  Value=0
  Sw_Indicator[0Stim|1Ext|2Mnv] : Constant  Value=2
  Indicator_State[] : Outport  VectorParamsAs1DForOutWhenUnconnected=off
  wires:
  ASM_OSI_Mapping/1(Indicator_State[]) -> Multiport Switch/4  "Mnv_Indicator_State[]"
  Stim_Indicator_State[]/1 -> Multiport Switch/2  "Stim_Indicator_State[]"
  Multiport Switch/1 -> Indicator_State[]/1  "Indicator_State[]"
  Saturation/1 -> Multiport Switch/1
  Rounding Function/1 -> Saturation/1
  Ext_Indicator_State[]/1 -> Multiport Switch/3  "Ext_Indicator_State[]"
  Fellow_TurnLights[]/1 -> ASM_OSI_Mapping/1(Fellow_TurnLights[])
  Sw_Indicator[0Stim|1Ext|2Mnv]/1 -> Rounding Function/1  "Sw_Indicator[0Stim|1Ext|2Mnv]"

== system ASM_Traffic_new/Environment/GroundTruth/UserInterface/PAR_Plant/Fellow_Vehicles/Lightstates_Fellow18/Indicator_State[] ==
  Fellow_TurnLights[] : Inport
  ASM_OSI_Mapping : Subsystem
  Ext_Indicator_State[] : Constant  Value=0
  Multiport Switch : MultiPortSwitch  DataPortOrder=Zero-based contiguous  zeroidx=on  SaturateOnIntegerOverflow=off  InputSameDT=off
  Rounding Function : Rounding  Operator=round
  Saturation : Saturate  UpperLimit=2  LowerLimit=0
  Stim_Indicator_State[] : Constant  Value=0
  Sw_Indicator[0Stim|1Ext|2Mnv] : Constant  Value=2
  Indicator_State[] : Outport  VectorParamsAs1DForOutWhenUnconnected=off
  wires:
  Sw_Indicator[0Stim|1Ext|2Mnv]/1 -> Rounding Function/1  "Sw_Indicator[0Stim|1Ext|2Mnv]"
  Fellow_TurnLights[]/1 -> ASM_OSI_Mapping/1(Fellow_TurnLights[])
  Ext_Indicator_State[]/1 -> Multiport Switch/3  "Ext_Indicator_State[]"
  Rounding Function/1 -> Saturation/1
  Saturation/1 -> Multiport Switch/1
  Multiport Switch/1 -> Indicator_State[]/1  "Indicator_State[]"
  Stim_Indicator_State[]/1 -> Multiport Switch/2  "Stim_Indicator_State[]"
  ASM_OSI_Mapping/1(Indicator_State[]) -> Multiport Switch/4  "Mnv_Indicator_State[]"

== system ASM_Traffic_new/Environment/GroundTruth/UserInterface/PAR_Plant/Fellow_Vehicles/Lightstates_Fellow19/Indicator_State[] ==
  Fellow_TurnLights[] : Inport
  ASM_OSI_Mapping : Subsystem
  Ext_Indicator_State[] : Constant  Value=0
  Multiport Switch : MultiPortSwitch  DataPortOrder=Zero-based contiguous  zeroidx=on  SaturateOnIntegerOverflow=off  InputSameDT=off
  Rounding Function : Rounding  Operator=round
  Saturation : Saturate  UpperLimit=2  LowerLimit=0
  Stim_Indicator_State[] : Constant  Value=0
  Sw_Indicator[0Stim|1Ext|2Mnv] : Constant  Value=2
  Indicator_State[] : Outport  VectorParamsAs1DForOutWhenUnconnected=off
  wires:
  ASM_OSI_Mapping/1(Indicator_State[]) -> Multiport Switch/4  "Mnv_Indicator_State[]"
  Stim_Indicator_State[]/1 -> Multiport Switch/2  "Stim_Indicator_State[]"
  Multiport Switch/1 -> Indicator_State[]/1  "Indicator_State[]"
  Saturation/1 -> Multiport Switch/1
  Rounding Function/1 -> Saturation/1
  Ext_Indicator_State[]/1 -> Multiport Switch/3  "Ext_Indicator_State[]"
  Fellow_TurnLights[]/1 -> ASM_OSI_Mapping/1(Fellow_TurnLights[])
  Sw_Indicator[0Stim|1Ext|2Mnv]/1 -> Rounding Function/1  "Sw_Indicator[0Stim|1Ext|2Mnv]"

== system ASM_Traffic_new/Environment/GroundTruth/UserInterface/PAR_Plant/Fellow_Vehicles/Lightstates_Fellow2/Indicator_State[] ==
  Fellow_TurnLights[] : Inport
  ASM_OSI_Mapping : Subsystem
  Ext_Indicator_State[] : Constant  Value=0
  Multiport Switch : MultiPortSwitch  DataPortOrder=Zero-based contiguous  zeroidx=on  SaturateOnIntegerOverflow=off  InputSameDT=off
  Rounding Function : Rounding  Operator=round
  Saturation : Saturate  UpperLimit=2  LowerLimit=0
  Stim_Indicator_State[] : Constant  Value=0
  Sw_Indicator[0Stim|1Ext|2Mnv] : Constant  Value=2
  Indicator_State[] : Outport  VectorParamsAs1DForOutWhenUnconnected=off
  wires:
  Sw_Indicator[0Stim|1Ext|2Mnv]/1 -> Rounding Function/1  "Sw_Indicator[0Stim|1Ext|2Mnv]"
  Fellow_TurnLights[]/1 -> ASM_OSI_Mapping/1(Fellow_TurnLights[])
  Ext_Indicator_State[]/1 -> Multiport Switch/3  "Ext_Indicator_State[]"
  Rounding Function/1 -> Saturation/1
  Saturation/1 -> Multiport Switch/1
  Multiport Switch/1 -> Indicator_State[]/1  "Indicator_State[]"
  Stim_Indicator_State[]/1 -> Multiport Switch/2  "Stim_Indicator_State[]"
  ASM_OSI_Mapping/1(Indicator_State[]) -> Multiport Switch/4  "Mnv_Indicator_State[]"

== system ASM_Traffic_new/Environment/GroundTruth/UserInterface/PAR_Plant/Fellow_Vehicles/Lightstates_Fellow20/Indicator_State[] ==
  Fellow_TurnLights[] : Inport
  ASM_OSI_Mapping : Subsystem
  Ext_Indicator_State[] : Constant  Value=0
  Multiport Switch : MultiPortSwitch  DataPortOrder=Zero-based contiguous  zeroidx=on  SaturateOnIntegerOverflow=off  InputSameDT=off
  Rounding Function : Rounding  Operator=round
  Saturation : Saturate  UpperLimit=2  LowerLimit=0
  Stim_Indicator_State[] : Constant  Value=0
  Sw_Indicator[0Stim|1Ext|2Mnv] : Constant  Value=2
  Indicator_State[] : Outport  VectorParamsAs1DForOutWhenUnconnected=off
  wires:
  Sw_Indicator[0Stim|1Ext|2Mnv]/1 -> Rounding Function/1  "Sw_Indicator[0Stim|1Ext|2Mnv]"
  Fellow_TurnLights[]/1 -> ASM_OSI_Mapping/1(Fellow_TurnLights[])
  Ext_Indicator_State[]/1 -> Multiport Switch/3  "Ext_Indicator_State[]"
  Rounding Function/1 -> Saturation/1
  Saturation/1 -> Multiport Switch/1
  Multiport Switch/1 -> Indicator_State[]/1  "Indicator_State[]"
  Stim_Indicator_State[]/1 -> Multiport Switch/2  "Stim_Indicator_State[]"
  ASM_OSI_Mapping/1(Indicator_State[]) -> Multiport Switch/4  "Mnv_Indicator_State[]"

== system ASM_Traffic_new/Environment/GroundTruth/UserInterface/PAR_Plant/Fellow_Vehicles/Lightstates_Fellow21/Indicator_State[] ==
  Fellow_TurnLights[] : Inport
  ASM_OSI_Mapping : Subsystem
  Ext_Indicator_State[] : Constant  Value=0
  Multiport Switch : MultiPortSwitch  DataPortOrder=Zero-based contiguous  zeroidx=on  SaturateOnIntegerOverflow=off  InputSameDT=off
  Rounding Function : Rounding  Operator=round
  Saturation : Saturate  UpperLimit=2  LowerLimit=0
  Stim_Indicator_State[] : Constant  Value=0
  Sw_Indicator[0Stim|1Ext|2Mnv] : Constant  Value=2
  Indicator_State[] : Outport  VectorParamsAs1DForOutWhenUnconnected=off
  wires:
  ASM_OSI_Mapping/1(Indicator_State[]) -> Multiport Switch/4  "Mnv_Indicator_State[]"
  Stim_Indicator_State[]/1 -> Multiport Switch/2  "Stim_Indicator_State[]"
  Multiport Switch/1 -> Indicator_State[]/1  "Indicator_State[]"
  Saturation/1 -> Multiport Switch/1
  Rounding Function/1 -> Saturation/1
  Ext_Indicator_State[]/1 -> Multiport Switch/3  "Ext_Indicator_State[]"
  Fellow_TurnLights[]/1 -> ASM_OSI_Mapping/1(Fellow_TurnLights[])
  Sw_Indicator[0Stim|1Ext|2Mnv]/1 -> Rounding Function/1  "Sw_Indicator[0Stim|1Ext|2Mnv]"

== system ASM_Traffic_new/Environment/GroundTruth/UserInterface/PAR_Plant/Fellow_Vehicles/Lightstates_Fellow22/Indicator_State[] ==
  Fellow_TurnLights[] : Inport
  ASM_OSI_Mapping : Subsystem
  Ext_Indicator_State[] : Constant  Value=0
  Multiport Switch : MultiPortSwitch  DataPortOrder=Zero-based contiguous  zeroidx=on  SaturateOnIntegerOverflow=off  InputSameDT=off
  Rounding Function : Rounding  Operator=round
  Saturation : Saturate  UpperLimit=2  LowerLimit=0
  Stim_Indicator_State[] : Constant  Value=0
  Sw_Indicator[0Stim|1Ext|2Mnv] : Constant  Value=2
  Indicator_State[] : Outport  VectorParamsAs1DForOutWhenUnconnected=off
  wires:
  Sw_Indicator[0Stim|1Ext|2Mnv]/1 -> Rounding Function/1  "Sw_Indicator[0Stim|1Ext|2Mnv]"
  Fellow_TurnLights[]/1 -> ASM_OSI_Mapping/1(Fellow_TurnLights[])
  Ext_Indicator_State[]/1 -> Multiport Switch/3  "Ext_Indicator_State[]"
  Rounding Function/1 -> Saturation/1
  Saturation/1 -> Multiport Switch/1
  Multiport Switch/1 -> Indicator_State[]/1  "Indicator_State[]"
  Stim_Indicator_State[]/1 -> Multiport Switch/2  "Stim_Indicator_State[]"
  ASM_OSI_Mapping/1(Indicator_State[]) -> Multiport Switch/4  "Mnv_Indicator_State[]"

== system ASM_Traffic_new/Environment/GroundTruth/UserInterface/PAR_Plant/Fellow_Vehicles/Lightstates_Fellow23/Indicator_State[] ==
  Fellow_TurnLights[] : Inport
  ASM_OSI_Mapping : Subsystem
  Ext_Indicator_State[] : Constant  Value=0
  Multiport Switch : MultiPortSwitch  DataPortOrder=Zero-based contiguous  zeroidx=on  SaturateOnIntegerOverflow=off  InputSameDT=off
  Rounding Function : Rounding  Operator=round
  Saturation : Saturate  UpperLimit=2  LowerLimit=0
  Stim_Indicator_State[] : Constant  Value=0
  Sw_Indicator[0Stim|1Ext|2Mnv] : Constant  Value=2
  Indicator_State[] : Outport  VectorParamsAs1DForOutWhenUnconnected=off
  wires:
  ASM_OSI_Mapping/1(Indicator_State[]) -> Multiport Switch/4  "Mnv_Indicator_State[]"
  Stim_Indicator_State[]/1 -> Multiport Switch/2  "Stim_Indicator_State[]"
  Multiport Switch/1 -> Indicator_State[]/1  "Indicator_State[]"
  Saturation/1 -> Multiport Switch/1
  Rounding Function/1 -> Saturation/1
  Ext_Indicator_State[]/1 -> Multiport Switch/3  "Ext_Indicator_State[]"
  Fellow_TurnLights[]/1 -> ASM_OSI_Mapping/1(Fellow_TurnLights[])
  Sw_Indicator[0Stim|1Ext|2Mnv]/1 -> Rounding Function/1  "Sw_Indicator[0Stim|1Ext|2Mnv]"

== system ASM_Traffic_new/Environment/GroundTruth/UserInterface/PAR_Plant/Fellow_Vehicles/Lightstates_Fellow24/Indicator_State[] ==
  Fellow_TurnLights[] : Inport
  ASM_OSI_Mapping : Subsystem
  Ext_Indicator_State[] : Constant  Value=0
  Multiport Switch : MultiPortSwitch  DataPortOrder=Zero-based contiguous  zeroidx=on  SaturateOnIntegerOverflow=off  InputSameDT=off
  Rounding Function : Rounding  Operator=round
  Saturation : Saturate  UpperLimit=2  LowerLimit=0
  Stim_Indicator_State[] : Constant  Value=0
  Sw_Indicator[0Stim|1Ext|2Mnv] : Constant  Value=2
  Indicator_State[] : Outport  VectorParamsAs1DForOutWhenUnconnected=off
  wires:
  Sw_Indicator[0Stim|1Ext|2Mnv]/1 -> Rounding Function/1  "Sw_Indicator[0Stim|1Ext|2Mnv]"
  Fellow_TurnLights[]/1 -> ASM_OSI_Mapping/1(Fellow_TurnLights[])
  Ext_Indicator_State[]/1 -> Multiport Switch/3  "Ext_Indicator_State[]"
  Rounding Function/1 -> Saturation/1
  Saturation/1 -> Multiport Switch/1
  Multiport Switch/1 -> Indicator_State[]/1  "Indicator_State[]"
  Stim_Indicator_State[]/1 -> Multiport Switch/2  "Stim_Indicator_State[]"
  ASM_OSI_Mapping/1(Indicator_State[]) -> Multiport Switch/4  "Mnv_Indicator_State[]"

== system ASM_Traffic_new/Environment/GroundTruth/UserInterface/PAR_Plant/Fellow_Vehicles/Lightstates_Fellow25/Indicator_State[] ==
  Fellow_TurnLights[] : Inport
  ASM_OSI_Mapping : Subsystem
  Ext_Indicator_State[] : Constant  Value=0
  Multiport Switch : MultiPortSwitch  DataPortOrder=Zero-based contiguous  zeroidx=on  SaturateOnIntegerOverflow=off  InputSameDT=off
  Rounding Function : Rounding  Operator=round
  Saturation : Saturate  UpperLimit=2  LowerLimit=0
  Stim_Indicator_State[] : Constant  Value=0
  Sw_Indicator[0Stim|1Ext|2Mnv] : Constant  Value=2
  Indicator_State[] : Outport  VectorParamsAs1DForOutWhenUnconnected=off
  wires:
  ASM_OSI_Mapping/1(Indicator_State[]) -> Multiport Switch/4  "Mnv_Indicator_State[]"
  Stim_Indicator_State[]/1 -> Multiport Switch/2  "Stim_Indicator_State[]"
  Multiport Switch/1 -> Indicator_State[]/1  "Indicator_State[]"
  Saturation/1 -> Multiport Switch/1
  Rounding Function/1 -> Saturation/1
  Ext_Indicator_State[]/1 -> Multiport Switch/3  "Ext_Indicator_State[]"
  Fellow_TurnLights[]/1 -> ASM_OSI_Mapping/1(Fellow_TurnLights[])
  Sw_Indicator[0Stim|1Ext|2Mnv]/1 -> Rounding Function/1  "Sw_Indicator[0Stim|1Ext|2Mnv]"

== system ASM_Traffic_new/Environment/GroundTruth/UserInterface/PAR_Plant/Fellow_Vehicles/Lightstates_Fellow26/Indicator_State[] ==
  Fellow_TurnLights[] : Inport
  ASM_OSI_Mapping : Subsystem
  Ext_Indicator_State[] : Constant  Value=0
  Multiport Switch : MultiPortSwitch  DataPortOrder=Zero-based contiguous  zeroidx=on  SaturateOnIntegerOverflow=off  InputSameDT=off
  Rounding Function : Rounding  Operator=round
  Saturation : Saturate  UpperLimit=2  LowerLimit=0
  Stim_Indicator_State[] : Constant  Value=0
  Sw_Indicator[0Stim|1Ext|2Mnv] : Constant  Value=2
  Indicator_State[] : Outport  VectorParamsAs1DForOutWhenUnconnected=off
  wires:
  Sw_Indicator[0Stim|1Ext|2Mnv]/1 -> Rounding Function/1  "Sw_Indicator[0Stim|1Ext|2Mnv]"
  Fellow_TurnLights[]/1 -> ASM_OSI_Mapping/1(Fellow_TurnLights[])
  Ext_Indicator_State[]/1 -> Multiport Switch/3  "Ext_Indicator_State[]"
  Rounding Function/1 -> Saturation/1
  Saturation/1 -> Multiport Switch/1
  Multiport Switch/1 -> Indicator_State[]/1  "Indicator_State[]"
  Stim_Indicator_State[]/1 -> Multiport Switch/2  "Stim_Indicator_State[]"
  ASM_OSI_Mapping/1(Indicator_State[]) -> Multiport Switch/4  "Mnv_Indicator_State[]"

== system ASM_Traffic_new/Environment/GroundTruth/UserInterface/PAR_Plant/Fellow_Vehicles/Lightstates_Fellow27/Indicator_State[] ==
  Fellow_TurnLights[] : Inport
  ASM_OSI_Mapping : Subsystem
  Ext_Indicator_State[] : Constant  Value=0
  Multiport Switch : MultiPortSwitch  DataPortOrder=Zero-based contiguous  zeroidx=on  SaturateOnIntegerOverflow=off  InputSameDT=off
  Rounding Function : Rounding  Operator=round
  Saturation : Saturate  UpperLimit=2  LowerLimit=0
  Stim_Indicator_State[] : Constant  Value=0
  Sw_Indicator[0Stim|1Ext|2Mnv] : Constant  Value=2
  Indicator_State[] : Outport  VectorParamsAs1DForOutWhenUnconnected=off
  wires:
  ASM_OSI_Mapping/1(Indicator_State[]) -> Multiport Switch/4  "Mnv_Indicator_State[]"
  Stim_Indicator_State[]/1 -> Multiport Switch/2  "Stim_Indicator_State[]"
  Multiport Switch/1 -> Indicator_State[]/1  "Indicator_State[]"
  Saturation/1 -> Multiport Switch/1
  Rounding Function/1 -> Saturation/1
  Ext_Indicator_State[]/1 -> Multiport Switch/3  "Ext_Indicator_State[]"
  Fellow_TurnLights[]/1 -> ASM_OSI_Mapping/1(Fellow_TurnLights[])
  Sw_Indicator[0Stim|1Ext|2Mnv]/1 -> Rounding Function/1  "Sw_Indicator[0Stim|1Ext|2Mnv]"

== system ASM_Traffic_new/Environment/GroundTruth/UserInterface/PAR_Plant/Fellow_Vehicles/Lightstates_Fellow28/Indicator_State[] ==
  Fellow_TurnLights[] : Inport
  ASM_OSI_Mapping : Subsystem
  Ext_Indicator_State[] : Constant  Value=0
  Multiport Switch : MultiPortSwitch  DataPortOrder=Zero-based contiguous  zeroidx=on  SaturateOnIntegerOverflow=off  InputSameDT=off
  Rounding Function : Rounding  Operator=round
  Saturation : Saturate  UpperLimit=2  LowerLimit=0
  Stim_Indicator_State[] : Constant  Value=0
  Sw_Indicator[0Stim|1Ext|2Mnv] : Constant  Value=2
  Indicator_State[] : Outport  VectorParamsAs1DForOutWhenUnconnected=off
  wires:
  Sw_Indicator[0Stim|1Ext|2Mnv]/1 -> Rounding Function/1  "Sw_Indicator[0Stim|1Ext|2Mnv]"
  Fellow_TurnLights[]/1 -> ASM_OSI_Mapping/1(Fellow_TurnLights[])
  Ext_Indicator_State[]/1 -> Multiport Switch/3  "Ext_Indicator_State[]"
  Rounding Function/1 -> Saturation/1
  Saturation/1 -> Multiport Switch/1
  Multiport Switch/1 -> Indicator_State[]/1  "Indicator_State[]"
  Stim_Indicator_State[]/1 -> Multiport Switch/2  "Stim_Indicator_State[]"
  ASM_OSI_Mapping/1(Indicator_State[]) -> Multiport Switch/4  "Mnv_Indicator_State[]"

== system ASM_Traffic_new/Environment/GroundTruth/UserInterface/PAR_Plant/Fellow_Vehicles/Lightstates_Fellow29/Indicator_State[] ==
  Fellow_TurnLights[] : Inport
  ASM_OSI_Mapping : Subsystem
  Ext_Indicator_State[] : Constant  Value=0
  Multiport Switch : MultiPortSwitch  DataPortOrder=Zero-based contiguous  zeroidx=on  SaturateOnIntegerOverflow=off  InputSameDT=off
  Rounding Function : Rounding  Operator=round
  Saturation : Saturate  UpperLimit=2  LowerLimit=0
  Stim_Indicator_State[] : Constant  Value=0
  Sw_Indicator[0Stim|1Ext|2Mnv] : Constant  Value=2
  Indicator_State[] : Outport  VectorParamsAs1DForOutWhenUnconnected=off
  wires:
  ASM_OSI_Mapping/1(Indicator_State[]) -> Multiport Switch/4  "Mnv_Indicator_State[]"
  Stim_Indicator_State[]/1 -> Multiport Switch/2  "Stim_Indicator_State[]"
  Multiport Switch/1 -> Indicator_State[]/1  "Indicator_State[]"
  Saturation/1 -> Multiport Switch/1
  Rounding Function/1 -> Saturation/1
  Ext_Indicator_State[]/1 -> Multiport Switch/3  "Ext_Indicator_State[]"
  Fellow_TurnLights[]/1 -> ASM_OSI_Mapping/1(Fellow_TurnLights[])
  Sw_Indicator[0Stim|1Ext|2Mnv]/1 -> Rounding Function/1  "Sw_Indicator[0Stim|1Ext|2Mnv]"

== system ASM_Traffic_new/Environment/GroundTruth/UserInterface/PAR_Plant/Fellow_Vehicles/Lightstates_Fellow3/Indicator_State[] ==
  Fellow_TurnLights[] : Inport
  ASM_OSI_Mapping : Subsystem
  Ext_Indicator_State[] : Constant  Value=0
  Multiport Switch : MultiPortSwitch  DataPortOrder=Zero-based contiguous  zeroidx=on  SaturateOnIntegerOverflow=off  InputSameDT=off
  Rounding Function : Rounding  Operator=round
  Saturation : Saturate  UpperLimit=2  LowerLimit=0
  Stim_Indicator_State[] : Constant  Value=0
  Sw_Indicator[0Stim|1Ext|2Mnv] : Constant  Value=2
  Indicator_State[] : Outport  VectorParamsAs1DForOutWhenUnconnected=off
  wires:
  ASM_OSI_Mapping/1(Indicator_State[]) -> Multiport Switch/4  "Mnv_Indicator_State[]"
  Stim_Indicator_State[]/1 -> Multiport Switch/2  "Stim_Indicator_State[]"
  Multiport Switch/1 -> Indicator_State[]/1  "Indicator_State[]"
  Saturation/1 -> Multiport Switch/1
  Rounding Function/1 -> Saturation/1
  Ext_Indicator_State[]/1 -> Multiport Switch/3  "Ext_Indicator_State[]"
  Fellow_TurnLights[]/1 -> ASM_OSI_Mapping/1(Fellow_TurnLights[])
  Sw_Indicator[0Stim|1Ext|2Mnv]/1 -> Rounding Function/1  "Sw_Indicator[0Stim|1Ext|2Mnv]"

== system ASM_Traffic_new/Environment/GroundTruth/UserInterface/PAR_Plant/Fellow_Vehicles/Lightstates_Fellow30/Indicator_State[] ==
  Fellow_TurnLights[] : Inport
  ASM_OSI_Mapping : Subsystem
  Ext_Indicator_State[] : Constant  Value=0
  Multiport Switch : MultiPortSwitch  DataPortOrder=Zero-based contiguous  zeroidx=on  SaturateOnIntegerOverflow=off  InputSameDT=off
  Rounding Function : Rounding  Operator=round
  Saturation : Saturate  UpperLimit=2  LowerLimit=0
  Stim_Indicator_State[] : Constant  Value=0
  Sw_Indicator[0Stim|1Ext|2Mnv] : Constant  Value=2
  Indicator_State[] : Outport  VectorParamsAs1DForOutWhenUnconnected=off
  wires:
  Sw_Indicator[0Stim|1Ext|2Mnv]/1 -> Rounding Function/1  "Sw_Indicator[0Stim|1Ext|2Mnv]"
  Fellow_TurnLights[]/1 -> ASM_OSI_Mapping/1(Fellow_TurnLights[])
  Ext_Indicator_State[]/1 -> Multiport Switch/3  "Ext_Indicator_State[]"
  Rounding Function/1 -> Saturation/1
  Saturation/1 -> Multiport Switch/1
  Multiport Switch/1 -> Indicator_State[]/1  "Indicator_State[]"
  Stim_Indicator_State[]/1 -> Multiport Switch/2  "Stim_Indicator_State[]"
  ASM_OSI_Mapping/1(Indicator_State[]) -> Multiport Switch/4  "Mnv_Indicator_State[]"

== system ASM_Traffic_new/Environment/GroundTruth/UserInterface/PAR_Plant/Fellow_Vehicles/Lightstates_Fellow4/Indicator_State[] ==
  Fellow_TurnLights[] : Inport
  ASM_OSI_Mapping : Subsystem
  Ext_Indicator_State[] : Constant  Value=0
  Multiport Switch : MultiPortSwitch  DataPortOrder=Zero-based contiguous  zeroidx=on  SaturateOnIntegerOverflow=off  InputSameDT=off
  Rounding Function : Rounding  Operator=round
  Saturation : Saturate  UpperLimit=2  LowerLimit=0
  Stim_Indicator_State[] : Constant  Value=0
  Sw_Indicator[0Stim|1Ext|2Mnv] : Constant  Value=2
  Indicator_State[] : Outport  VectorParamsAs1DForOutWhenUnconnected=off
  wires:
  Sw_Indicator[0Stim|1Ext|2Mnv]/1 -> Rounding Function/1  "Sw_Indicator[0Stim|1Ext|2Mnv]"
  Fellow_TurnLights[]/1 -> ASM_OSI_Mapping/1(Fellow_TurnLights[])
  Ext_Indicator_State[]/1 -> Multiport Switch/3  "Ext_Indicator_State[]"
  Rounding Function/1 -> Saturation/1
  Saturation/1 -> Multiport Switch/1
  Multiport Switch/1 -> Indicator_State[]/1  "Indicator_State[]"
  Stim_Indicator_State[]/1 -> Multiport Switch/2  "Stim_Indicator_State[]"
  ASM_OSI_Mapping/1(Indicator_State[]) -> Multiport Switch/4  "Mnv_Indicator_State[]"

== system ASM_Traffic_new/Environment/GroundTruth/UserInterface/PAR_Plant/Fellow_Vehicles/Lightstates_Fellow5/Indicator_State[] ==
  Fellow_TurnLights[] : Inport
  ASM_OSI_Mapping : Subsystem
  Ext_Indicator_State[] : Constant  Value=0
  Multiport Switch : MultiPortSwitch  DataPortOrder=Zero-based contiguous  zeroidx=on  SaturateOnIntegerOverflow=off  InputSameDT=off
  Rounding Function : Rounding  Operator=round
  Saturation : Saturate  UpperLimit=2  LowerLimit=0
  Stim_Indicator_State[] : Constant  Value=0
  Sw_Indicator[0Stim|1Ext|2Mnv] : Constant  Value=2
  Indicator_State[] : Outport  VectorParamsAs1DForOutWhenUnconnected=off
  wires:
  ASM_OSI_Mapping/1(Indicator_State[]) -> Multiport Switch/4  "Mnv_Indicator_State[]"
  Stim_Indicator_State[]/1 -> Multiport Switch/2  "Stim_Indicator_State[]"
  Multiport Switch/1 -> Indicator_State[]/1  "Indicator_State[]"
  Saturation/1 -> Multiport Switch/1
  Rounding Function/1 -> Saturation/1
  Ext_Indicator_State[]/1 -> Multiport Switch/3  "Ext_Indicator_State[]"
  Fellow_TurnLights[]/1 -> ASM_OSI_Mapping/1(Fellow_TurnLights[])
  Sw_Indicator[0Stim|1Ext|2Mnv]/1 -> Rounding Function/1  "Sw_Indicator[0Stim|1Ext|2Mnv]"

== system ASM_Traffic_new/Environment/GroundTruth/UserInterface/PAR_Plant/Fellow_Vehicles/Lightstates_Fellow6/Indicator_State[] ==
  Fellow_TurnLights[] : Inport
  ASM_OSI_Mapping : Subsystem
  Ext_Indicator_State[] : Constant  Value=0
  Multiport Switch : MultiPortSwitch  DataPortOrder=Zero-based contiguous  zeroidx=on  SaturateOnIntegerOverflow=off  InputSameDT=off
  Rounding Function : Rounding  Operator=round
  Saturation : Saturate  UpperLimit=2  LowerLimit=0
  Stim_Indicator_State[] : Constant  Value=0
  Sw_Indicator[0Stim|1Ext|2Mnv] : Constant  Value=2
  Indicator_State[] : Outport  VectorParamsAs1DForOutWhenUnconnected=off
  wires:
  Sw_Indicator[0Stim|1Ext|2Mnv]/1 -> Rounding Function/1  "Sw_Indicator[0Stim|1Ext|2Mnv]"
  Fellow_TurnLights[]/1 -> ASM_OSI_Mapping/1(Fellow_TurnLights[])
  Ext_Indicator_State[]/1 -> Multiport Switch/3  "Ext_Indicator_State[]"
  Rounding Function/1 -> Saturation/1
  Saturation/1 -> Multiport Switch/1
  Multiport Switch/1 -> Indicator_State[]/1  "Indicator_State[]"
  Stim_Indicator_State[]/1 -> Multiport Switch/2  "Stim_Indicator_State[]"
  ASM_OSI_Mapping/1(Indicator_State[]) -> Multiport Switch/4  "Mnv_Indicator_State[]"
